simulink model "yig_tuning_model"  (R2026b)
settings: Solver=FixedStepDiscrete  StopTime=Tstop  FixedStep=Ts
InitFcn:
  | if ~exist('YIG','var') || ~exist('ref_profile','var'), yig_setup; end
values from neighbouring files (symbols this model uses):
  Tc = YIG.sim.Tc    [yig_setup.m]
  Ts = YIG.sim.Ts    [yig_setup.m]
settings Model: Creator=Fairret  LastModifiedBy=Fairret
settings DataIOCC: SaveOutput=off  SaveTime=off

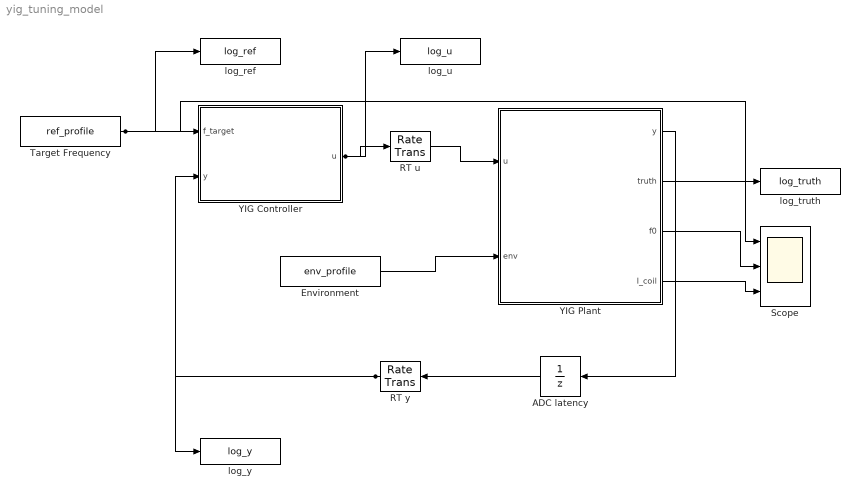
== system yig_tuning_model ==
  ADC latency : UnitDelay  SampleTime=Ts
  Environment : FromWorkspace  VariableName=env_profile  SampleTime=Ts  OutputAfterFinalValue=Holding final value
  RT u : RateTransition  OutPortSampleTime=Ts
  RT y : RateTransition  OutPortSampleTime=Tc
  Scope : Scope  NumInputPorts=3
  Target Frequency : FromWorkspace  VariableName=ref_profile  SampleTime=Tc  Interpolate=off  OutputAfterFinalValue=Holding final value
  YIG Controller : MATLAB Function  TreatAsAtomicUnit=on
      settings: AttributesFormatString=edit: control\yig_controller.m
  YIG Plant : Subsystem
      settings: AttributesFormatString=params: YIG = yig_params()
  log_ref : ToWorkspace  VariableName=log_ref  SaveFormat=Timeseries  SampleTime=-1
  log_truth : ToWorkspace  VariableName=log_truth  SaveFormat=Timeseries  SampleTime=-1
      settings: Decimation=YIG.sim.log_decim
  log_u : ToWorkspace  VariableName=log_u  SaveFormat=Timeseries  SampleTime=-1
  log_y : ToWorkspace  VariableName=log_y  SaveFormat=Timeseries  SampleTime=-1
  wires:
  Target Frequency/1 -> YIG Controller/1(f_target), log_ref/1, Scope/1
  YIG Controller/1(u) -> RT u/1, log_u/1
  RT u/1 -> YIG Plant/1(u)
  Environment/1 -> YIG Plant/2(env)
  YIG Plant/1(y) -> ADC latency/1
  ADC latency/1 -> RT y/1
  RT y/1 -> YIG Controller/2(y), log_y/1
  YIG Plant/2(truth) -> log_truth/1
  YIG Plant/3(f0) -> Scope/2
  YIG Plant/4(I_coil) -> Scope/3

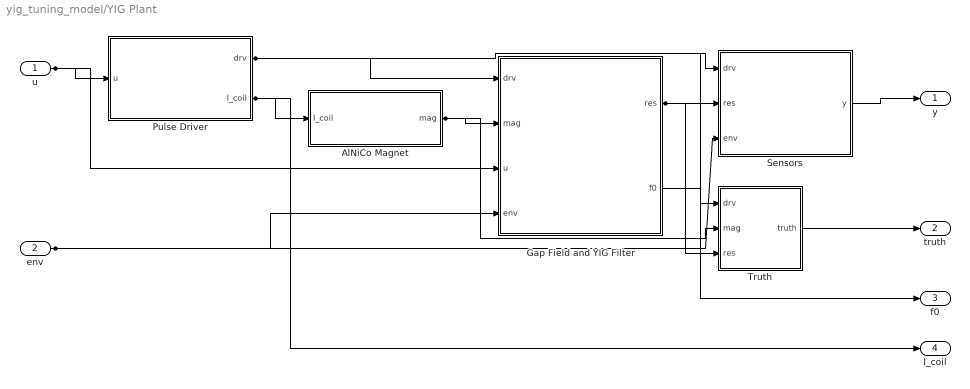
== system yig_tuning_model/YIG Plant ==
  u : Inport
  env : Inport  Port=2
  AlNiCo Magnet : MATLAB Function  TreatAsAtomicUnit=on
  Gap Field and YIG Filter : MATLAB Function  TreatAsAtomicUnit=on
  Pulse Driver : MATLAB Function  TreatAsAtomicUnit=on
  Sensors : MATLAB Function  TreatAsAtomicUnit=on
  Truth : MATLAB Function  TreatAsAtomicUnit=on
  y : Outport
  truth : Outport  Port=2
  f0 : Outport  Port=3
  I_coil : Outport  Port=4
  wires:
  u/1 -> Pulse Driver/1(u), Gap Field and YIG Filter/3(u)
  env/1 -> Gap Field and YIG Filter/4(env), Sensors/3(env)
  Pulse Driver/1(drv) -> Gap Field and YIG Filter/1(drv), Sensors/1(drv), Truth/1(drv)
  Pulse Driver/2(I_coil) -> AlNiCo Magnet/1(I_coil), I_coil/1
  AlNiCo Magnet/1(mag) -> Gap Field and YIG Filter/2(mag), Truth/2(mag)
  Gap Field and YIG Filter/1(res) -> Sensors/2(res), Truth/3(res)
  Gap Field and YIG Filter/2(f0) -> f0/1
  Sensors/1(y) -> y/1
  Truth/1(truth) -> truth/1

== matlab function yig_tuning_model/YIG Plant/Pulse Driver ==
  data: u input; drv output size=[5 1]; I_coil output size=1; YIG parameter
function [drv, I_coil] = fcn(u, YIG)
%#codegen
% Charger + cap + H-bridge + main coil + trim coil.  See plant/yig_driver_step.m
% drv = [I_coil; Vc; busy; ready; I_trim]
drv = yig_driver_step(u, YIG);
I_coil = drv(1);

== matlab function yig_tuning_model/YIG Controller ==
  data: f_target input; u output size=[6 1]; y input; YIG parameter
function u = fcn(f_target, y, YIG)
%#codegen
% YIG Controller block.
% This is only a wrapper -- put your control law in control/yig_controller.m
% (or change the line below to call a different function with the
%  same signature:  u = my_ctrl(f_target, y, YIG) ).
%   f_target : desired centre frequency [Hz]
%   y (8x1)  : measurements, see yig_sensors_step.m
%   u (6x1)  : [V0_set; fire; polarity; I_lim; I_trim; f_probe]
u = yig_controller(f_target, y, YIG);

== matlab function yig_tuning_model/YIG Plant/AlNiCo Magnet ==
  data: I_coil input; mag output size=[3 1]; YIG parameter
function mag = fcn(I_coil, YIG)
%#codegen
% Preisach hysteresis + self-demag.  See plant/yig_magnet_step.m
% mag = [m; H_eff; H_coil]
mag = yig_magnet_step(I_coil, YIG);

== matlab function yig_tuning_model/YIG Plant/Gap Field and YIG Filter ==
  data: drv input; mag input; u input; res output size=[3 1]; env input; f0 output size=1; YIG parameter
function [res, f0] = fcn(drv, mag, u, env, YIG)
%#codegen
% Gap field -> YIG resonance -> filter response.  See plant/yig_resonator_step.m
% res = [f0; B_gap; P_out_dBm]
res = yig_resonator_step(drv, mag, u, env, YIG);
f0 = res(1);

== matlab function yig_tuning_model/YIG Plant/Sensors ==
  data: drv input; y output size=[8 1]; res input; env input; YIG parameter
function y = fcn(drv, res, env, YIG)
%#codegen
% Noisy, quantised measurements.  See plant/yig_sensors_step.m
y = yig_sensors_step(drv, res, env, YIG);

== matlab function yig_tuning_model/YIG Plant/Truth ==
  data: drv input; truth output size=[11 1]; mag input; res input; YIG parameter
function truth = fcn(drv, mag, res, YIG)
%#codegen
% Logged plant states: [drv(5); mag(3); res(3)]
truth = [drv(:); mag(:); res(:)];
